simulink model "des_supervisor"  (R2026b)
settings: Solver=FixedStepDiscrete  StopTime=inf  FixedStep=0.01
PreLoadFcn:
  | addpath(fullfile(fileparts(fileparts(which('des_supervisor'))), 'src'));
settings Model: Creator=yecha  LastModifiedBy=yecha
settings HardwareCC: ProdHWDeviceType=ARM Compatible->ARM 64-bit (LP64)  ProdLargestAtomicFloat=Double  ProdLargestAtomicInteger=LongLong  ProdLongLongMode=on
settings RTWCC: GenCodeOnly=on  RTWVerbose=off
settings GRTTargetCC: MatFileLogging=off  SupportNonFinite=off

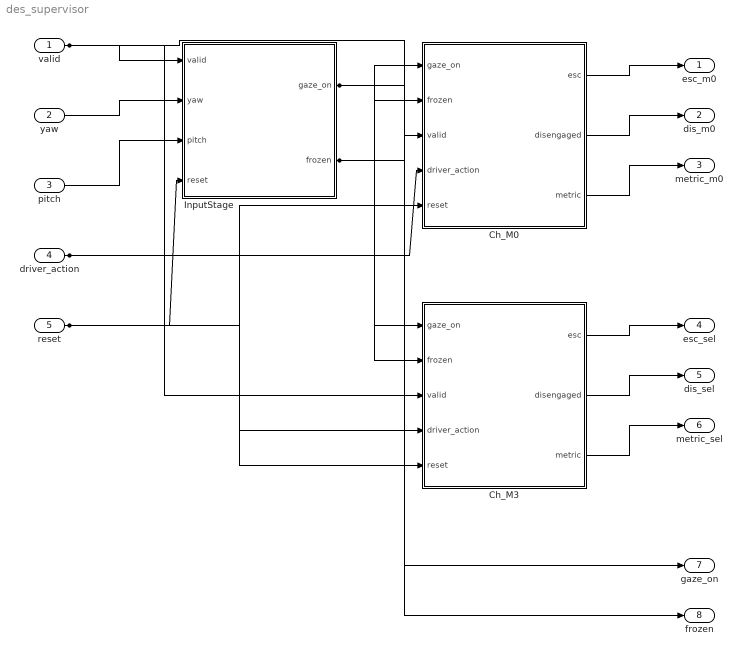
== system des_supervisor ==
  valid : Inport  OutDataTypeStr=boolean  PortDimensions=1  SampleTime=0.01  Interpolate=off
  yaw : Inport  Port=2  OutDataTypeStr=double  PortDimensions=1  SampleTime=0.01  Interpolate=off
  pitch : Inport  Port=3  OutDataTypeStr=double  PortDimensions=1  SampleTime=0.01  Interpolate=off
  driver_action : Inport  Port=4  OutDataTypeStr=boolean  PortDimensions=1  SampleTime=0.01  Interpolate=off
  reset : Inport  Port=5  OutDataTypeStr=boolean  PortDimensions=1  SampleTime=0.01  Interpolate=off
  Ch_M0 : Subsystem
  Ch_M3 : Subsystem
  InputStage : MATLAB Function  TreatAsAtomicUnit=on
  esc_m0 : Outport
  dis_m0 : Outport  Port=2
  metric_m0 : Outport  Port=3
  esc_sel : Outport  Port=4
  dis_sel : Outport  Port=5
  metric_sel : Outport  Port=6
  gaze_on : Outport  Port=7
  frozen : Outport  Port=8
  wires:
  valid/1 -> InputStage/1(valid), Ch_M0/3(valid), Ch_M3/3(valid)
  yaw/1 -> InputStage/2(yaw)
  pitch/1 -> InputStage/3(pitch)
  reset/1 -> InputStage/4(reset), Ch_M0/5(reset), Ch_M3/5(reset)
  InputStage/1(gaze_on) -> Ch_M0/1(gaze_on), Ch_M3/1(gaze_on), gaze_on/1
  InputStage/2(frozen) -> Ch_M0/2(frozen), Ch_M3/2(frozen), frozen/1
  driver_action/1 -> Ch_M0/4(driver_action), Ch_M3/4(driver_action)
  Ch_M0/1(esc) -> esc_m0/1
  Ch_M0/2(disengaged) -> dis_m0/1
  Ch_M0/3(metric) -> metric_m0/1
  Ch_M3/1(esc) -> esc_sel/1
  Ch_M3/2(disengaged) -> dis_sel/1
  Ch_M3/3(metric) -> metric_sel/1

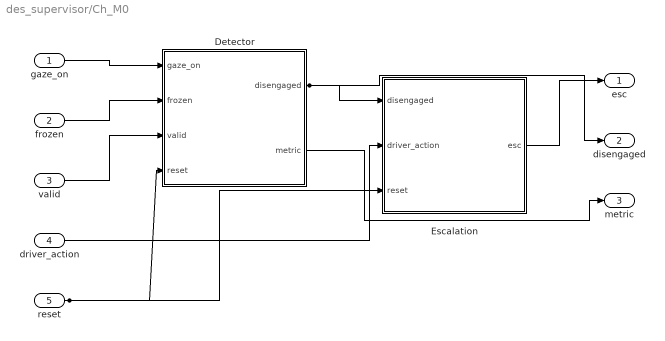
== system des_supervisor/Ch_M0 ==
  gaze_on : Inport
  frozen : Inport  Port=2
  valid : Inport  Port=3
  driver_action : Inport  Port=4
  reset : Inport  Port=5
  Detector : MATLAB Function  TreatAsAtomicUnit=on
  Escalation : Stateflow chart  TreatAsAtomicUnit=on
  esc : Outport
  disengaged : Outport  Port=2
  metric : Outport  Port=3
  wires:
  gaze_on/1 -> Detector/1(gaze_on)
  frozen/1 -> Detector/2(frozen)
  valid/1 -> Detector/3(valid)
  reset/1 -> Detector/4(reset), Escalation/3(reset)
  Detector/1(disengaged) -> Escalation/1(disengaged), disengaged/1
  driver_action/1 -> Escalation/2(driver_action)
  Escalation/1(esc) -> esc/1
  Detector/2(metric) -> metric/1

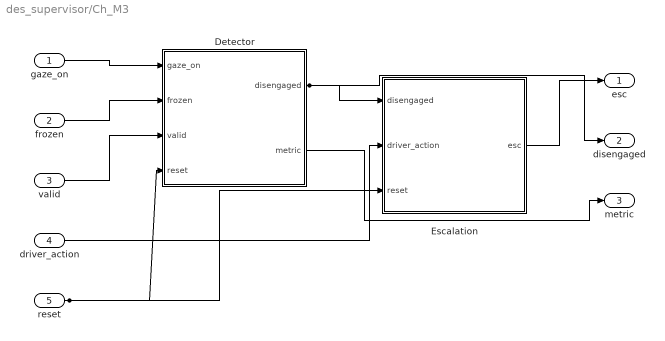
== system des_supervisor/Ch_M3 ==
  gaze_on : Inport
  frozen : Inport  Port=2
  valid : Inport  Port=3
  driver_action : Inport  Port=4
  reset : Inport  Port=5
  Detector : MATLAB Function  TreatAsAtomicUnit=on
  Escalation : Stateflow chart  TreatAsAtomicUnit=on
  esc : Outport
  disengaged : Outport  Port=2
  metric : Outport  Port=3
  wires:
  gaze_on/1 -> Detector/1(gaze_on)
  frozen/1 -> Detector/2(frozen)
  valid/1 -> Detector/3(valid)
  reset/1 -> Detector/4(reset), Escalation/3(reset)
  Detector/1(disengaged) -> Escalation/1(disengaged), disengaged/1
  driver_action/1 -> Escalation/2(driver_action)
  Escalation/1(esc) -> esc/1
  Detector/2(metric) -> metric/1

== matlab function des_supervisor/Ch_M0/Detector ==
  data: gaze_on input; disengaged output; frozen input; valid input; reset input; metric output
function [disengaged, metric] = Detector(gaze_on, frozen, valid, reset)
% 감지 계층 M0 (src/des_detect.m). R171 기본 타이머 OR 모델별 판정
P = des_params(0);
persistent S
if isempty(S)
    S = des_init(P);
end
if reset
    S = des_init(P);
end
v = valid && ~(P.fz_enable && frozen);   % 고정(사진) 의심이면 미검출과 같게 처리
[S, disengaged, ~, metric] = des_detect(S, gaze_on, v, P);

== matlab function des_supervisor/InputStage ==
  data: valid input; gaze_on output; yaw input; pitch input; reset input; frozen output
function [gaze_on, frozen] = InputStage(valid, yaw, pitch, reset)
% 입력 단계: 주시 영역 판정 + 고정 탐지 (src/des_input_step.m)
P = des_params(3);
persistent SI
if isempty(SI)
    SI = des_input_init(P);
end
if reset
    SI = des_input_init(P);
end
[SI, gaze_on, frozen] = des_input_step(SI, valid, yaw, pitch, P);

== stateflow chart des_supervisor/Ch_M0/Escalation ==
  settings: updateMethod=DISCRETE  sampleTime=0.01  executeAtInitialization=1
  state ENGAGED
    entry: esc = uint8(0);
  state EOR
    entry: esc = uint8(1);
  state EOR_ENH
    entry: esc = uint8(2);
  state DCA
    entry: esc = uint8(3);
  state UNAVAILABLE
    entry: esc = uint8(4);
  (default) -> ENGAGED
  ENGAGED -> EOR : [disengaged]
  EOR -> EOR_ENH [order 2] : after(300, tick)
  EOR_ENH -> DCA [order 2] : after(500, tick)
  DCA -> UNAVAILABLE [order 2] : after(500, tick)
  EOR -> ENGAGED [order 1] : [reset || ~disengaged]
  EOR_ENH -> ENGAGED [order 1] : [reset || ~disengaged]
  DCA -> ENGAGED [order 1] : [reset || (~disengaged && driver_action)]
  UNAVAILABLE -> ENGAGED : [reset]
  data: disengaged input boolean; driver_action input boolean; reset input boolean; esc output uint8

== matlab function des_supervisor/Ch_M3/Detector ==
  data: gaze_on input; disengaged output; frozen input; valid input; reset input; metric output
function [disengaged, metric] = Detector(gaze_on, frozen, valid, reset)
% 감지 계층 M3 (src/des_detect.m). R171 기본 타이머 OR 모델별 판정
P = des_params(3);
persistent S
if isempty(S)
    S = des_init(P);
end
if reset
    S = des_init(P);
end
v = valid && ~(P.fz_enable && frozen);   % 고정(사진) 의심이면 미검출과 같게 처리
[S, disengaged, ~, metric] = des_detect(S, gaze_on, v, P);

== stateflow chart des_supervisor/Ch_M3/Escalation ==
  settings: updateMethod=DISCRETE  sampleTime=0.01  executeAtInitialization=1
  state ENGAGED
    entry: esc = uint8(0);
  state EOR
    entry: esc = uint8(1);
  state EOR_ENH
    entry: esc = uint8(2);
  state DCA
    entry: esc = uint8(3);
  state UNAVAILABLE
    entry: esc = uint8(4);
  (default) -> ENGAGED
  ENGAGED -> EOR : [disengaged]
  EOR -> EOR_ENH [order 2] : after(300, tick)
  EOR_ENH -> DCA [order 2] : after(500, tick)
  DCA -> UNAVAILABLE [order 2] : after(500, tick)
  EOR -> ENGAGED [order 1] : [reset || ~disengaged]
  EOR_ENH -> ENGAGED [order 1] : [reset || ~disengaged]
  DCA -> ENGAGED [order 1] : [reset || (~disengaged && driver_action)]
  UNAVAILABLE -> ENGAGED : [reset]
  data: disengaged input boolean; driver_action input boolean; reset input boolean; esc output uint8
